simulink model "CW_bangbangantry"  (R2025b)
settings: Solver=FixedStepAuto  StartTime=0.0  StopTime=inf  FixedStep=0.005  RelTol=1e-3  EnableMultiTasking=on
model workspace (MAT data in the model file):
  Movethresh = 2
  Stopthresh = 1
libraries: raspberrypiBasiclib x5, simulink x1, raspberrypiNetworklib x1
settings Model: ExtModeTrigDuration=2  Creator=ioannisgeorgilas  LastModifiedBy=Lenovo ThinkPad
settings SolverCC: PositivePriorityOrder=on
settings OptimizationCC: EnhancedBackFolding=on  PassReuseOutputArgsAs=Individual arguments  ZeroExternalMemoryAtStartup=off  ZeroInternalMemoryAtStartup=off  MaxStackSize=200000  OptimizeBlockOrder=speed  DifferentSizesBufferReuse=on  OptimizationCustomize=off  EfficientTunableParamExpr=on
settings DebuggingCC: ParameterTunabilityLossMsg=error
settings HardwareCC: ProdBitPerPointer=32.0  ProdBitPerSizeT=32.0  ProdBitPerPtrDiffT=32.0  ProdLargestAtomicInteger=Long  ProdLargestAtomicFloat=Double  ProdWordSize=32.0  ProdLongLongMode=on  ProdHWDeviceType=ARM Compatible->ARM Cortex-A (32-bit)
settings RTWCC: SystemTargetFile=ert.tlc  HardwareBoard=Raspberry Pi  TLCOptions="-aInlineSetEventsForThisBaseRateFcn=TLC_FALSE -aSuppressMultiTaskScheduler=TLC_FALSE  -aRateBasedStepFcn=0"  TemplateMakefile=ert_default_tmf  Toolchain=GNU GCC Embedded Linux  BuildConfiguration=Faster Runs  Description=Embedded Coder
settings CodeAppCC: ForceParamTrailComments=on  IgnoreCustomStorageClasses=off  OperatorAnnotations=on  SimulinkDataObjDesc=on  SFDataObjDesc=on  InsertBlockDesc=on
settings ERTTargetCC: ExtModeTransport=2.0  ExtModeStaticAlloc=on  ExtModeMexFile=ext_xcp  ExtModeIntrfLevel=Level2 - Open  InlinedParameterPlacement=Hierarchical  CodeReplacementLibrary=ARM Cortex-A CMSIS  SupportVariableSizeSignals=on

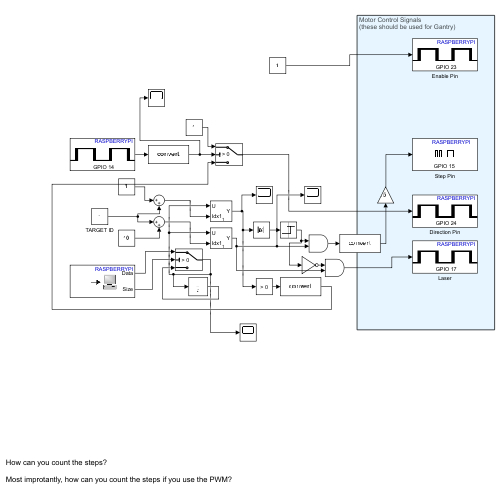
[thumbnail: Simulink's stored preview of the top-level diagram]
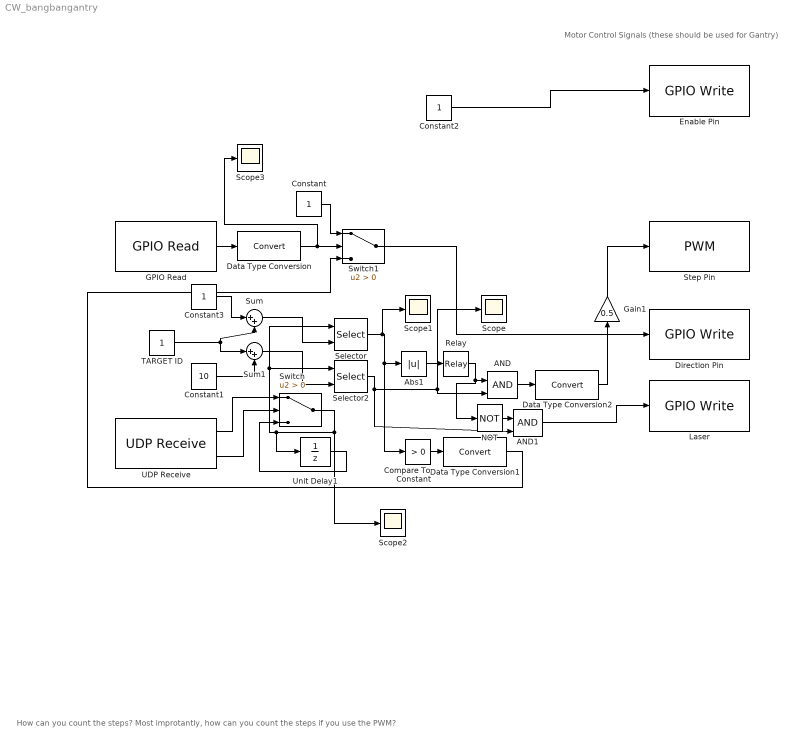
== system CW_bangbangantry ==
  note: How can you count the steps?
      |
      | Most improtantly, how can you count the steps if you use the PWM?
  note: Motor Control Signals
      | (these should be used for Gantry)
  AND : Logic  IconShape=distinctive  AllPortsSameDT=off  OutDataTypeStr=boolean
  AND1 : Logic  IconShape=distinctive  AllPortsSameDT=off  OutDataTypeStr=boolean
  Abs1 : Abs  SaturateOnIntegerOverflow=off
  Compare To Constant : simulink/Logic and Bit Operations/Compare To Constant  relop=>  const=0  OutDataTypeStr=boolean
  Constant : Constant
  Constant1 : Constant  Value=10
  Constant2 : Constant
  Constant3 : Constant
  Data Type Conversion : DataTypeConversion  SaturateOnIntegerOverflow=off  RndMeth=Floor
  Data Type Conversion1 : DataTypeConversion  SaturateOnIntegerOverflow=off  RndMeth=Floor
  Data Type Conversion2 : DataTypeConversion  SaturateOnIntegerOverflow=off  RndMeth=Floor
  Direction Pin : raspberrypiBasiclib/GPIO Write  BoardProperty=Pi 3 Model B+  gpio=24  blockPlatform=Raspberry Pi  PinNumber=17  board=[]  direction=[]
  Enable Pin : raspberrypiBasiclib/GPIO Write  BoardProperty=Pi 3 Model B+  gpio=23  blockPlatform=Raspberry Pi  PinNumber=17  board=[]  direction=[]
  GPIO Read : raspberrypiBasiclib/GPIO Read  BoardProperty=Pi 3 Model B+  gpio=14  SampleTime=-1  blockPlatform=Raspberry Pi  PinNumber=4  board=[]  direction=[]  internalResistor=[]
  Gain1 : Gain  Gain=0.5
  Laser : raspberrypiBasiclib/GPIO Write  BoardProperty=Pi 4 Model B  gpio=17  blockPlatform=Raspberry Pi  PinNumber=17  board=[]  direction=[]
  NOT : Logic  Operator=NOT  IconShape=distinctive  AllPortsSameDT=off  OutDataTypeStr=boolean
  Relay : Relay  OnSwitchValue=Movethresh  OffSwitchValue=Stopthresh
  Scope{,1..3} (4 alike) : Scope
      Scope2 settings: DataLoggingVariableName=ScopeData2
      Scope3 settings: DataLoggingVariableName=ScopeData3
  Selector : Selector  InputPortWidth=20  IndexOptions=Index vector (port)  Indices=[1 3]  OutputSizes=1
  Selector2 : Selector  InputPortWidth=20  IndexOptions=Index vector (port)  Indices=[1 3]  OutputSizes=1
  Step Pin : raspberrypiBasiclib/PWM  board=Pi 3 Model B+  Pin_=15  Frequency=100  blockPlatform=Raspberry Pi
  Sum : Sum  Inputs=|++
  Sum1 : Sum  Inputs=|++
  Switch : Switch  Criteria=u2 > Threshold  SaturateOnIntegerOverflow=off  InputSameDT=off
  Switch1 : Switch  Criteria=u2 > Threshold  SaturateOnIntegerOverflow=off  InputSameDT=off
  TARGET ID : Constant
  UDP Receive : raspberrypiNetworklib/UDP Receive  localURL='0.0.0.0'  localPort=5005  remoteURL='0.0.0.0'  remotePort=-1  recvBufferSize=8192  signalDatatype=double  dims=2  isVarSize=off  showBlockingTime=off  blockingTime=0  sampletime=0.01  blockPlatform=Raspberry Pi
  Unit Delay1 : UnitDelay  InitialCondition=zeros(20,1)  SampleTime=-1  HasFrameUpgradeWarning=on
  wires:
  UDP Receive/1 -> Switch/1
  UDP Receive/2 -> Switch/2
  Unit Delay1/1 -> Switch/3
  Switch/1 -> Scope2/1, Selector2/1, Selector/1, Unit Delay1/1
  Selector2/1 -> AND1/2, Scope/1, AND/2
  Abs1/1 -> Relay/1
  Relay/1 -> NOT/1, AND/1
  NOT/1 -> AND1/1
  AND/1 -> Data Type Conversion2/1
  Data Type Conversion2/1 -> Gain1/1
  Compare To Constant/1 -> Data Type Conversion1/1
  AND1/1 -> Laser/1
  Constant2/1 -> Enable Pin/1
  GPIO Read/1 -> Data Type Conversion/1
  Data Type Conversion/1 -> Scope3/1, Switch1/2
  Data Type Conversion1/1 -> Switch1/3
  Constant/1 -> Switch1/1
  Switch1/1 -> Direction Pin/1
  Gain1/1 -> Step Pin/1
  TARGET ID/1 -> Sum/2, Sum1/1
  Sum1/1 -> Selector2/2
  Constant1/1 -> Sum1/2
  Selector/1 -> Scope1/1, Compare To Constant/1, Abs1/1
  Constant3/1 -> Sum/1
  Sum/1 -> Selector/2
